simulink model "edge_pipeline_latency"  (R2026b)
settings: Solver=ode45  StopTime=1  MaxStep=0.0005
settings Model: Creator=rithvin007  LastModifiedBy=rithvin007

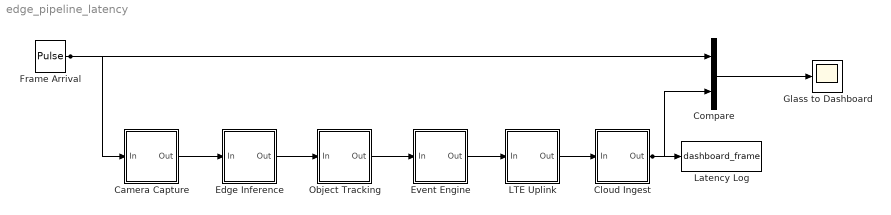
== system edge_pipeline_latency ==
  Camera Capture : Subsystem
  Cloud Ingest : Subsystem
  Compare : Mux  Inputs=2
  Edge Inference : Subsystem
  Event Engine : Subsystem
  Frame Arrival : DiscretePulseGenerator  PulseType=Time based  Period=0.0333  PulseWidth=20
  Glass to Dashboard : Scope
  LTE Uplink : Subsystem
  Latency Log : ToWorkspace  VariableName=dashboard_frame  SaveFormat=Timeseries  SampleTime=-1
  Object Tracking : Subsystem
  wires:
  Cloud Ingest/1(Out) -> Latency Log/1, Compare/2
  Event Engine/1(Out) -> LTE Uplink/1(In)
  Compare/1 -> Glass to Dashboard/1
  Object Tracking/1(Out) -> Event Engine/1(In)
  Edge Inference/1(Out) -> Object Tracking/1(In)
  LTE Uplink/1(Out) -> Cloud Ingest/1(In)
  Camera Capture/1(Out) -> Edge Inference/1(In)
  Frame Arrival/1 -> Camera Capture/1(In), Compare/1

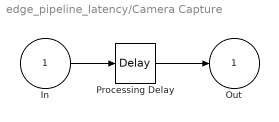
== system edge_pipeline_latency/Camera Capture ==
  In : Inport
  Processing Delay : TransportDelay  DelayTime=0.005
  Out : Outport
  wires:
  Processing Delay/1 -> Out/1
  In/1 -> Processing Delay/1

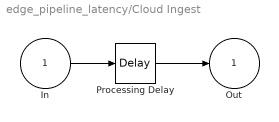
== system edge_pipeline_latency/Cloud Ingest ==
  In : Inport
  Processing Delay : TransportDelay  DelayTime=0.012
  Out : Outport
  wires:
  Processing Delay/1 -> Out/1
  In/1 -> Processing Delay/1

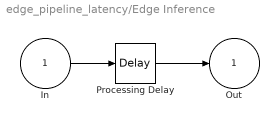
== system edge_pipeline_latency/Edge Inference ==
  In : Inport
  Processing Delay : TransportDelay  DelayTime=0.022
  Out : Outport
  wires:
  Processing Delay/1 -> Out/1
  In/1 -> Processing Delay/1

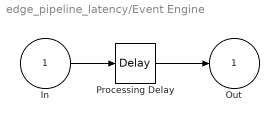
== system edge_pipeline_latency/Event Engine ==
  In : Inport
  Processing Delay : TransportDelay  DelayTime=0.002
  Out : Outport
  wires:
  Processing Delay/1 -> Out/1
  In/1 -> Processing Delay/1

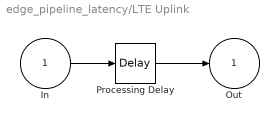
== system edge_pipeline_latency/LTE Uplink ==
  In : Inport
  Processing Delay : TransportDelay  DelayTime=0.085
  Out : Outport
  wires:
  Processing Delay/1 -> Out/1
  In/1 -> Processing Delay/1

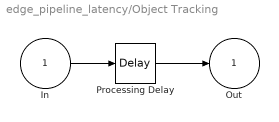
== system edge_pipeline_latency/Object Tracking ==
  In : Inport
  Processing Delay : TransportDelay  DelayTime=0.004
  Out : Outport
  wires:
  Processing Delay/1 -> Out/1
  In/1 -> Processing Delay/1
